simulink model "travail3_exo2"  (R2016a)
settings: Solver=VariableStepAuto  StartTime=0.0  StopTime=250  RelTol=1e-3
settings Model: Creator=KONE MOHAMED  LastModifiedBy=KONE MOHAMED

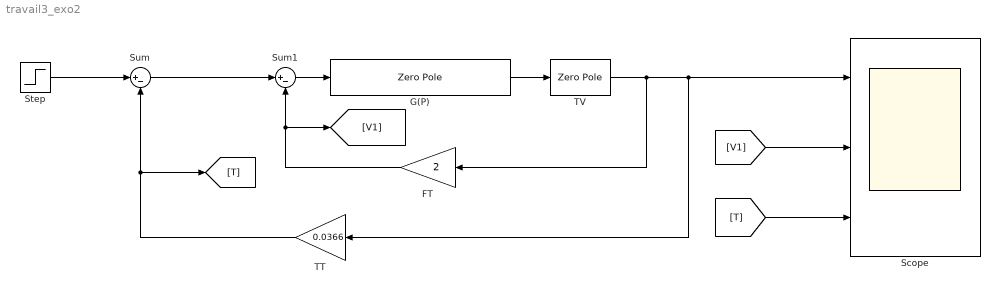
== system travail3_exo2 ==
  "FT " : Gain  Gain=2
  G(P) : ZeroPole  Zeros=[]  Poles=[-1/10 -1/10]  Gain=[0.15]
  Scope : Scope  NumInputPorts=3
  Step : Step  After=90/60  SampleTime=0
  Sum : Sum  Inputs=|+-
  Sum1 : Sum  Inputs=|+-
  "TT " : Gain  Gain=0.0366
  TV : ZeroPole  Zeros=[]  Poles=[-1/5]  Gain=[2]
  wires:
  TV/1 -> "FT "/1, "TT "/1, Scope/1
  "FT "/1 -> Sum1/2, [V1]
  Sum/1 -> Sum1/1
  Sum1/1 -> G(P)/1
  "TT "/1 -> [T], Sum/2
  G(P)/1 -> TV/1
  Step/1 -> Sum/1
  [V1] -> Scope/2
  [T] -> Scope/3
